simulink library "AFCToolbox2023a"  (R2023a)
settings: Solver=VariableStepAuto  StartTime=0.0  StopTime=10.0  RelTol=1e-3
undefined symbols (not defined in the file or in its folder): AFC5Toolbox_SimuMoudle, AFCToolbox, ax, ay, az, btnSample, C_d, C_dm, C_m, C_t, Control, d, declination_table, dp0, dp1, dp2, dp3, dt, euler_0, g0, I_xyz, inclination_table, J_m, lmd_high, lmd_low, lp_acc_knoise, lp_acc_max, lp_acc_min, lp_acc_seed, lp_GPS_BL_max, lp_GPS_BL_min, lp_GPS_H_max, lp_GPS_H_min, lp_GPS_knoise, lp_GPS_seed, lp_GPS_vel_max, lp_GPS_vel_min, lp_gyro_knoise, lp_gyro_max, lp_gyro_min, lp_gyro_seed, lp_hf_vwind, lp_hs_vwind_interp, lp_kaerorho, lp_kaeroT, lp_kIxyz, lp_kmass, lp_momentx_A0, lp_momentx_Af, lp_momentx_ts, lp_momenty_A0, lp_momenty_Af, lp_momenty_ts, lp_momentz_A0, lp_momentz_Af, lp_momentz_ts, lp_vf_vwind, lp_vs_vwind_interp, lp_vwind_thetax, lp_vwind_thetaz ... (+54)
libraries: $bdroot x104, simulink x75, etargetslib x32, sharedtransform x13, simulink_extras x12, dspstat3 x11, aerolibconvert2 x9, aerolibtransform2 x3, aerolibutil x2, matrix_library x1
(part 7 of 10)

== system AFCToolbox2023a/SimuMoudle/Forces & Moments1/Parameters/Air Parameter1/Air Model/Pressure xishu ==
  note: 9
  note: 1
  note: 2
  note: 3
  note: 4
  note: 5
  note: 6
  note: 7
  note: 8
  Z : Inport
  H : Inport  Port=2
  1 : Switch  Threshold=11.0191  SaturateOnIntegerOverflow=off  InputSameDT=off
  2 : Switch  Threshold=20.0631  SaturateOnIntegerOverflow=off  InputSameDT=off
  3 : Switch  Threshold=32.1619  SaturateOnIntegerOverflow=off  InputSameDT=off
  4 : Switch  Threshold=47.3501  SaturateOnIntegerOverflow=off  InputSameDT=off
  5 : Switch  Threshold=51.4125  SaturateOnIntegerOverflow=off  InputSameDT=off
  6 : Switch  Threshold=71.8020  SaturateOnIntegerOverflow=off  InputSameDT=off
  7 : Switch  Threshold=86  SaturateOnIntegerOverflow=off  InputSameDT=off
  8 : Switch  Threshold=91  SaturateOnIntegerOverflow=off  InputSameDT=off
  Gain : Gain  Gain=1.042e-3
  Gain1 : Gain  Gain=1e-6
  Sum : Sum  Inputs=|++
  constant1 : Constant  Value=2.1671e-4
  constant10 : Constant  Value=8.9155e-4
  constant11 : Constant  Value=2.8338e-3
  constant2 : Constant  Value=0
  constant4 : Constant  Value=1.2274e-5
  constant6 : Constant  Value=2.2730
  constant7 : Constant
  constant8 : Constant  Value=1.1953e-1
  constant9 : Constant  Value=2.5158e-2
  xishu : Outport
  wires:
  Gain1/1 -> 7/1
  Gain/1 -> Sum/2
  H/1 -> Gain/1
  Sum/1 -> Gain1/1
  constant6/1 -> Sum/1
  8/1 -> xishu/1
  7/1 -> 8/3
  constant2/1 -> 8/1
  constant7/1 -> 1/3
  constant8/1 -> 1/1
  constant9/1 -> 2/1
  1/1 -> 2/3
  constant11/1 -> 3/1
  2/1 -> 3/3
  constant10/1 -> 4/1
  3/1 -> 4/3
  constant1/1 -> 5/1
  4/1 -> 5/3
  constant4/1 -> 6/1
  5/1 -> 6/3
  6/1 -> 7/3
  Z/1 -> 2/2, 8/2, 7/2, 6/2, 5/2, 1/2, 3/2, 4/2

== system AFCToolbox2023a/SimuMoudle/Forces & Moments1/Parameters/Air Parameter1/Air Model/T ==
  note: 1
  note: 2
  note: 3
  note: 4
  note: 5
  note: 6
  note: 7
  note: 8
  Z : Inport
  T xishu : Inport  Port=2
  W : Inport  Port=3
  1 : Switch  Threshold=11.0191  SaturateOnIntegerOverflow=off  InputSameDT=off
  2 : Switch  Threshold=20.0631  SaturateOnIntegerOverflow=off  InputSameDT=off
  3 : Switch  Threshold=32.1619  SaturateOnIntegerOverflow=off  InputSameDT=off
  4 : Switch  Threshold=47.3501  SaturateOnIntegerOverflow=off  InputSameDT=off
  5 : Switch  Threshold=51.4125  SaturateOnIntegerOverflow=off  InputSameDT=off
  6 : Switch  Threshold=71.8020  SaturateOnIntegerOverflow=off  InputSameDT=off
  7 : Switch  Threshold=86  SaturateOnIntegerOverflow=off  InputSameDT=off
  Product : Product  RndMeth=Zero
  constant10 : Constant
  constant6 : Constant
  constant8 : Constant
  T : Outport
  wires:
  Product/1 -> T/1
  T xishu/1 -> Product/2
  7/1 -> Product/1
  W/1 -> 3/1, 2/1, 5/1, 6/1, 1/3
  constant8/1 -> 1/1
  1/1 -> 2/3
  2/1 -> 3/3
  constant10/1 -> 4/1
  3/1 -> 4/3
  4/1 -> 5/3
  5/1 -> 6/3
  constant6/1 -> 7/1
  6/1 -> 7/3
  Z/1 -> 2/2, 6/2, 7/2, 5/2, 1/2, 3/2, 4/2

== system AFCToolbox2023a/SimuMoudle/Forces & Moments1/Parameters/Air Parameter1/Air Model/T xishu ==
  note: 8
  note: 7
  note: 6
  note: 5
  note: 4
  note: 3
  note: 2
  note: 1
  Z : Inport
  1 : Switch  Threshold=11.0191  SaturateOnIntegerOverflow=off  InputSameDT=off
  2 : Switch  Threshold=20.0631  SaturateOnIntegerOverflow=off  InputSameDT=off
  3 : Switch  Threshold=32.1619  SaturateOnIntegerOverflow=off  InputSameDT=off
  4 : Switch  Threshold=47.3501  SaturateOnIntegerOverflow=off  InputSameDT=off
  5 : Switch  Threshold=51.4125  SaturateOnIntegerOverflow=off  InputSameDT=off
  6 : Switch  Threshold=71.8020  SaturateOnIntegerOverflow=off  InputSameDT=off
  7 : Switch  Threshold=86  SaturateOnIntegerOverflow=off  InputSameDT=off
  constant1 : Constant  Value=247.021
  constant10 : Constant  Value=270.650
  constant11 : Constant  Value=250.350
  constant4 : Constant  Value=200.590
  constant6 : Constant  Value=186.870
  constant7 : Constant  Value=288.15
  constant8 : Constant  Value=216.650
  constant9 : Constant  Value=221.552
  T xishu : Outport
  wires:
  7/1 -> T xishu/1
  Z/1 -> 4/2, 3/2, 1/2, 5/2, 7/2, 6/2, 2/2
  6/1 -> 7/3
  constant6/1 -> 7/1
  5/1 -> 6/3
  constant4/1 -> 6/1
  4/1 -> 5/3
  constant1/1 -> 5/1
  3/1 -> 4/3
  constant10/1 -> 4/1
  2/1 -> 3/3
  constant11/1 -> 3/1
  1/1 -> 2/3
  constant9/1 -> 2/1
  constant8/1 -> 1/1
  constant7/1 -> 1/3

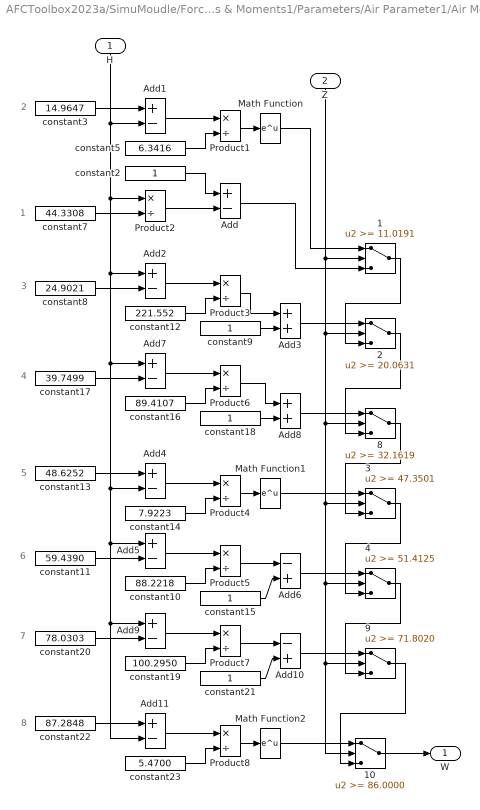
== system AFCToolbox2023a/SimuMoudle/Forces & Moments1/Parameters/Air Parameter1/Air Model/W ==
  note: 8
  note: 7
  note: 4
  note: 6
  note: 5
  note: 3
  note: 2
  note: 1
  H : Inport
  Z : Inport  Port=2
  1 : Switch  Threshold=11.0191  SaturateOnIntegerOverflow=off  InputSameDT=off
  10 : Switch  Threshold=86.0000  SaturateOnIntegerOverflow=off  InputSameDT=off
  2 : Switch  Threshold=20.0631  SaturateOnIntegerOverflow=off  InputSameDT=off
  3 : Switch  Threshold=47.3501  SaturateOnIntegerOverflow=off  InputSameDT=off
  4 : Switch  Threshold=51.4125  SaturateOnIntegerOverflow=off  InputSameDT=off
  8 : Switch  Threshold=32.1619  SaturateOnIntegerOverflow=off  InputSameDT=off
  9 : Switch  Threshold=71.8020  SaturateOnIntegerOverflow=off  InputSameDT=off
  Add{,1..2,4..5,7,9,11} (8 alike) : Sum  Inputs=+-
  Add10 : Sum  Inputs=-+
  Add3 : Sum  Inputs=2
  Add6 : Sum  Inputs=-+
  Add8 : Sum  Inputs=2
  Math Function : Math  SignedPower=on
  Math Function1 : Math  SignedPower=on
  Math Function2 : Math  SignedPower=on
  Product{1..8} (8 alike) : Product  Inputs=*/  RndMeth=Zero
  constant10 : Constant  Value=88.2218
  constant11 : Constant  Value=59.4390
  constant12 : Constant  Value=221.552
  constant13 : Constant  Value=48.6252
  constant14 : Constant  Value=7.9223
  constant{2,9,15,18,21} (5 alike) : Constant
  constant16 : Constant  Value=89.4107
  constant17 : Constant  Value=39.7499
  constant19 : Constant  Value=100.2950
  constant20 : Constant  Value=78.0303
  constant22 : Constant  Value=87.2848
  constant23 : Constant  Value=5.4700
  constant3 : Constant  Value=14.9647
  constant5 : Constant  Value=6.3416
  constant7 : Constant  Value=44.3308
  constant8 : Constant  Value=24.9021
  W : Outport
  wires:
  Z/1 -> 1/2, 2/2, 8/2, 3/2, 4/2, 9/2, 10/2
  10/1 -> W/1
  9/1 -> 10/3
  constant22/1 -> Add11/1
  Math Function2/1 -> 10/1
  Product8/1 -> Math Function2/1
  constant23/1 -> Product8/2
  Add11/1 -> Product8/1
  Add10/1 -> 9/1
  constant21/1 -> Add10/2
  Product7/1 -> Add10/1
  constant20/1 -> Add9/2
  constant19/1 -> Product7/2
  Add9/1 -> Product7/1
  4/1 -> 9/3
  Add7/1 -> Product6/1
  8/1 -> 3/3
  Add8/1 -> 8/1
  constant18/1 -> Add8/2
  Product6/1 -> Add8/1
  constant17/1 -> Add7/2
  constant16/1 -> Product6/2
  2/1 -> 8/3
  Add6/1 -> 4/1
  constant15/1 -> Add6/2
  Product5/1 -> Add6/1
  constant11/1 -> Add5/2
  constant10/1 -> Product5/2
  Add5/1 -> Product5/1
  Math Function1/1 -> 3/1
  Product4/1 -> Math Function1/1
  constant14/1 -> Product4/2
  Add4/1 -> Product4/1
  constant13/1 -> Add4/1
  Add3/1 -> 2/1
  constant9/1 -> Add3/2
  Product3/1 -> Add3/1
  constant8/1 -> Add2/2
  constant12/1 -> Product3/2
  Add2/1 -> Product3/1
  Math Function/1 -> 1/1
  Product1/1 -> Math Function/1
  constant5/1 -> Product1/2
  Add1/1 -> Product1/1
  constant3/1 -> Add1/1
  Product2/1 -> Add/2
  constant2/1 -> Add/1
  constant7/1 -> Product2/2
  Add/1 -> 1/3
  1/1 -> 2/3
  3/1 -> 4/3
  H/1 -> Add7/1, Add11/2, Add9/1, Add5/1, Add4/2, Add2/1, Product2/1, Add1/2

== system AFCToolbox2023a/SimuMoudle/Forces & Moments1/Parameters/Air Parameter1/Air Model/W zhishu ==
  note: 1
  note: 2
  note: 3
  note: 4
  note: 5
  note: 6
  note: 7
  note: 8
  Z : Inport
  1 : Switch  Threshold=11.0191  SaturateOnIntegerOverflow=off  InputSameDT=off
  2 : Switch  Threshold=20.0631  SaturateOnIntegerOverflow=off  InputSameDT=off
  3 : Switch  Threshold=32.1619  SaturateOnIntegerOverflow=off  InputSameDT=off
  4 : Switch  Threshold=47.3501  SaturateOnIntegerOverflow=off  InputSameDT=off
  5 : Switch  Threshold=51.4125  SaturateOnIntegerOverflow=off  InputSameDT=off
  6 : Switch  Threshold=71.8020  SaturateOnIntegerOverflow=off  InputSameDT=off
  7 : Switch  Threshold=86  SaturateOnIntegerOverflow=off  InputSameDT=off
  constant1 : Constant  Value=11.2011
  constant10 : Constant
  constant11 : Constant  Value=-13.2011
  constant4 : Constant  Value=16.0816
  constant6 : Constant
  constant7 : Constant  Value=4.2559
  constant8 : Constant
  constant9 : Constant  Value=-35.1629
  zhishu : Outport
  wires:
  constant7/1 -> 1/3
  constant8/1 -> 1/1
  constant9/1 -> 2/1
  1/1 -> 2/3
  constant11/1 -> 3/1
  2/1 -> 3/3
  constant10/1 -> 4/1
  3/1 -> 4/3
  constant1/1 -> 5/1
  4/1 -> 5/3
  constant4/1 -> 6/1
  5/1 -> 6/3
  constant6/1 -> 7/1
  6/1 -> 7/3
  Z/1 -> 2/2, 6/2, 7/2, 5/2, 1/2, 3/2, 4/2
  7/1 -> zhishu/1

== system AFCToolbox2023a/SimuMoudle/Forces & Moments1/Parameters/Air Parameter1/Air Model/W zhishu1 ==
  note: 8
  note: 7
  note: 6
  note: 5
  note: 4
  note: 3
  note: 2
  note: 1
  Z : Inport
  1 : Switch  Threshold=11.0191  SaturateOnIntegerOverflow=off  InputSameDT=off
  2 : Switch  Threshold=20.0631  SaturateOnIntegerOverflow=off  InputSameDT=off
  3 : Switch  Threshold=32.1619  SaturateOnIntegerOverflow=off  InputSameDT=off
  4 : Switch  Threshold=47.3501  SaturateOnIntegerOverflow=off  InputSameDT=off
  5 : Switch  Threshold=51.4125  SaturateOnIntegerOverflow=off  InputSameDT=off
  6 : Switch  Threshold=71.8020  SaturateOnIntegerOverflow=off  InputSameDT=off
  7 : Switch  Threshold=86  SaturateOnIntegerOverflow=off  InputSameDT=off
  constant1 : Constant  Value=12.2011
  constant10 : Constant
  constant11 : Constant  Value=-12.2011
  constant4 : Constant  Value=17.0816
  constant6 : Constant
  constant7 : Constant  Value=5.2559
  constant8 : Constant
  constant9 : Constant  Value=-34.1629
  zhishu : Outport
  wires:
  7/1 -> zhishu/1
  Z/1 -> 4/2, 3/2, 1/2, 5/2, 7/2, 6/2, 2/2
  6/1 -> 7/3
  constant6/1 -> 7/1
  5/1 -> 6/3
  constant4/1 -> 6/1
  4/1 -> 5/3
  constant1/1 -> 5/1
  3/1 -> 4/3
  constant10/1 -> 4/1
  2/1 -> 3/3
  constant11/1 -> 3/1
  1/1 -> 2/3
  constant9/1 -> 2/1
  constant8/1 -> 1/1
  constant7/1 -> 1/3

== system AFCToolbox2023a/SimuMoudle/Forces & Moments1/Parameters/Air Parameter1/Air Model/rho xishu ==
  note: 8
  note: 7
  note: 6
  note: 5
  note: 4
  note: 3
  note: 2
  note: 1
  note: 9
  Z : Inport
  1 : Switch  Threshold=11.0191  SaturateOnIntegerOverflow=off  InputSameDT=off
  2 : Switch  Threshold=20.0631  SaturateOnIntegerOverflow=off  InputSameDT=off
  3 : Switch  Threshold=32.1619  SaturateOnIntegerOverflow=off  InputSameDT=off
  4 : Switch  Threshold=47.3501  SaturateOnIntegerOverflow=off  InputSameDT=off
  5 : Switch  Threshold=51.4125  SaturateOnIntegerOverflow=off  InputSameDT=off
  6 : Switch  Threshold=71.8020  SaturateOnIntegerOverflow=off  InputSameDT=off
  7 : Switch  Threshold=86  SaturateOnIntegerOverflow=off  InputSameDT=off
  8 : Switch  Threshold=91  SaturateOnIntegerOverflow=off  InputSameDT=off
  constant1 : Constant  Value=2.5280e-4
  constant10 : Constant  Value=9.4920e-4
  constant11 : Constant  Value=3.2618e-3
  constant2 : Constant  Value=0
  constant4 : Constant  Value=1.7632e-5
  constant6 : Constant  Value=3.6411e-6
  constant7 : Constant
  constant8 : Constant  Value=1.5898e-1
  constant9 : Constant  Value=3.2722e-2
  xishu : Outport
  wires:
  Z/1 -> 4/2, 3/2, 1/2, 5/2, 6/2, 7/2, 8/2, 2/2
  6/1 -> 7/3
  constant6/1 -> 7/1
  5/1 -> 6/3
  constant4/1 -> 6/1
  4/1 -> 5/3
  constant1/1 -> 5/1
  3/1 -> 4/3
  constant10/1 -> 4/1
  2/1 -> 3/3
  constant11/1 -> 3/1
  1/1 -> 2/3
  constant9/1 -> 2/1
  constant8/1 -> 1/1
  constant7/1 -> 1/3
  constant2/1 -> 8/1
  7/1 -> 8/3
  8/1 -> xishu/1

== system AFCToolbox2023a/SimuMoudle/Position-Control/Leader/Subsystem/Follower1/Subsystem ==
  v111_k_1 : Inport
  v000_k_1 : Inport  Port=2
  Abs : Abs  SaturateOnIntegerOverflow=off
  Abs1 : Abs  SaturateOnIntegerOverflow=off
  Abs2 : Abs  SaturateOnIntegerOverflow=off
  Add : Sum  Inputs=+-
  Add1 : Sum  Inputs=+-
  Add2 : Sum  Inputs=+-
  Demux : Demux  Outputs=3
  Demux1 : Demux  Outputs=3
  Max : MinMax  Function=max  Inputs=3
  Relational Operator : RelationalOperator  Operator=>  OutDataTypeStr=boolean  RndMeth=Simplest  InputSameDT=off
  get lmd : Subsystem
  order : Outport
  wires:
  Relational Operator/1 -> order/1
  get lmd/1(lmd) -> Relational Operator/2
  Max/1 -> Relational Operator/1
  Abs2/1 -> Max/3
  Abs1/1 -> Max/2
  Abs/1 -> Max/1
  Add2/1 -> Abs2/1
  Add1/1 -> Abs1/1
  Add/1 -> Abs/1
  Demux/3 -> Add2/1
  Demux1/3 -> Add2/2
  Demux1/2 -> Add1/2
  Demux/2 -> Add1/1
  Demux1/1 -> Add/2
  Demux/1 -> Add/1
  v000_k_1/1 -> Demux1/1
  v111_k_1/1 -> Demux/1

== system AFCToolbox2023a/SimuMoudle/Position-Control/Leader/Subsystem/Follower1/Subsystem1 ==
  Clock : Clock
  Constant : Constant
  Constant1 : Constant  Value=0
  Switch1 : Switch  Criteria=u2 > Threshold  Threshold=40  SaturateOnIntegerOverflow=off  InputSameDT=off
  Out1 : Outport
  wires:
  Switch1/1 -> Out1/1
  Constant1/1 -> Switch1/3
  Constant/1 -> Switch1/1
  Clock/1 -> Switch1/2

== system AFCToolbox2023a/SimuMoudle/Position-Control/Leader/Subsystem/Follower1/质心运动方程 ==
  v1 : Inport
  theta1 : Inport  Port=2
  phi1 : Inport  Port=3
  Enable : EnablePort
  Cos : Trigonometry  Operator=cos
  Cos1 : Trigonometry  Operator=cos
  Mux : Mux  Inputs=3
  Product : Product  Inputs=3
  Product1 : Product  Inputs=3
  Product2 : Product
  Sin : Trigonometry
  Sin1 : Trigonometry
  v111 : Outport
  wires:
  theta1/1 -> Cos/1, Sin/1
  phi1/1 -> Cos1/1, Sin1/1
  Cos/1 -> Product/1
  v1/1 -> Product2/2, Product1/3, Product/3
  Product/1 -> Mux/1
  Product1/1 -> Mux/2
  Sin/1 -> Product1/1
  Cos1/1 -> Product/2, Product1/2
  Product2/1 -> Mux/3
  Mux/1 -> v111/1
  Sin1/1 -> Product2/1

== system AFCToolbox2023a/SimuMoudle/Position-Control/Leader/Subsystem/Follower2/Subsystem ==
  v222_k_1 : Inport
  v000_k_1 : Inport  Port=2
  Abs : Abs  SaturateOnIntegerOverflow=off
  Abs1 : Abs  SaturateOnIntegerOverflow=off
  Abs2 : Abs  SaturateOnIntegerOverflow=off
  Add : Sum  Inputs=+-
  Add1 : Sum  Inputs=+-
  Add2 : Sum  Inputs=+-
  Demux : Demux  Outputs=3
  Demux1 : Demux  Outputs=3
  Max : MinMax  Function=max  Inputs=3
  Relational Operator : RelationalOperator  Operator=>  OutDataTypeStr=boolean  RndMeth=Simplest  InputSameDT=off
  get lmd : Subsystem
  order : Outport
  wires:
  v222_k_1/1 -> Demux/1
  v000_k_1/1 -> Demux1/1
  Demux/1 -> Add/1
  Demux1/1 -> Add/2
  Demux/2 -> Add1/1
  Demux1/2 -> Add1/2
  Demux1/3 -> Add2/2
  Demux/3 -> Add2/1
  Add/1 -> Abs/1
  Add1/1 -> Abs1/1
  Add2/1 -> Abs2/1
  Abs/1 -> Max/1
  Abs1/1 -> Max/2
  Abs2/1 -> Max/3
  Max/1 -> Relational Operator/1
  get lmd/1(lmd) -> Relational Operator/2
  Relational Operator/1 -> order/1

== system AFCToolbox2023a/SimuMoudle/Position-Control/Leader/Subsystem/Follower2/Subsystem1 ==
  Clock : Clock
  Constant : Constant
  Constant1 : Constant  Value=0
  Switch1 : Switch  Criteria=u2 > Threshold  Threshold=40  SaturateOnIntegerOverflow=off  InputSameDT=off
  Out1 : Outport
  wires:
  Switch1/1 -> Out1/1
  Constant1/1 -> Switch1/3
  Constant/1 -> Switch1/1
  Clock/1 -> Switch1/2

== system AFCToolbox2023a/SimuMoudle/Position-Control/Leader/Subsystem/Follower2/质心运动方程 ==
  v2 : Inport
  theta2 : Inport  Port=2
  phi2 : Inport  Port=3
  Enable : EnablePort
  Cos : Trigonometry  Operator=cos
  Cos1 : Trigonometry  Operator=cos
  Mux : Mux  Inputs=3
  Product : Product  Inputs=3
  Product1 : Product  Inputs=3
  Product2 : Product
  Sin : Trigonometry
  Sin1 : Trigonometry
  v222 : Outport
  wires:
  Sin1/1 -> Product2/1
  Mux/1 -> v222/1
  Product2/1 -> Mux/3
  Cos1/1 -> Product1/2, Product/2
  Sin/1 -> Product1/1
  Product1/1 -> Mux/2
  Product/1 -> Mux/1
  v2/1 -> Product/3, Product1/3, Product2/2
  Cos/1 -> Product/1
  phi2/1 -> Sin1/1, Cos1/1
  theta2/1 -> Sin/1, Cos/1

== system AFCToolbox2023a/SimuMoudle/Position-Control/Leader/Subsystem/Follower3/Subsystem ==
  v333_k_1 : Inport
  v000_k_1 : Inport  Port=2
  Abs : Abs  SaturateOnIntegerOverflow=off
  Abs1 : Abs  SaturateOnIntegerOverflow=off
  Abs2 : Abs  SaturateOnIntegerOverflow=off
  Add : Sum  Inputs=+-
  Add1 : Sum  Inputs=+-
  Add2 : Sum  Inputs=+-
  Demux : Demux  Outputs=3
  Demux1 : Demux  Outputs=3
  Max : MinMax  Function=max  Inputs=3
  Relational Operator : RelationalOperator  Operator=>  OutDataTypeStr=boolean  RndMeth=Simplest  InputSameDT=off
  get lmd : Subsystem
  order : Outport
  wires:
  Relational Operator/1 -> order/1
  get lmd/1(lmd) -> Relational Operator/2
  Max/1 -> Relational Operator/1
  Abs2/1 -> Max/3
  Abs1/1 -> Max/2
  Abs/1 -> Max/1
  Add2/1 -> Abs2/1
  Add1/1 -> Abs1/1
  Add/1 -> Abs/1
  Demux/3 -> Add2/1
  Demux1/3 -> Add2/2
  Demux1/2 -> Add1/2
  Demux/2 -> Add1/1
  Demux1/1 -> Add/2
  Demux/1 -> Add/1
  v000_k_1/1 -> Demux1/1
  v333_k_1/1 -> Demux/1

== system AFCToolbox2023a/SimuMoudle/Position-Control/Leader/Subsystem/Follower3/Subsystem1 ==
  Clock : Clock
  Constant : Constant
  Constant1 : Constant  Value=0
  Switch1 : Switch  Criteria=u2 > Threshold  Threshold=40  SaturateOnIntegerOverflow=off  InputSameDT=off
  Out1 : Outport
  wires:
  Switch1/1 -> Out1/1
  Constant1/1 -> Switch1/3
  Constant/1 -> Switch1/1
  Clock/1 -> Switch1/2

== system AFCToolbox2023a/SimuMoudle/Position-Control/Leader/Subsystem/Follower3/质心运动方程 ==
  v3 : Inport
  theta3 : Inport  Port=2
  phi3 : Inport  Port=3
  Enable : EnablePort
  Cos : Trigonometry  Operator=cos
  Cos1 : Trigonometry  Operator=cos
  Mux : Mux  Inputs=3
  Product : Product  Inputs=3
  Product1 : Product  Inputs=3
  Product2 : Product
  Sin : Trigonometry
  Sin1 : Trigonometry
  v333 : Outport
  wires:
  theta3/1 -> Cos/1, Sin/1
  phi3/1 -> Cos1/1, Sin1/1
  Cos/1 -> Product/1
  v3/1 -> Product2/2, Product1/3, Product/3
  Product/1 -> Mux/1
  Product1/1 -> Mux/2
  Sin/1 -> Product1/1
  Cos1/1 -> Product/2, Product1/2
  Product2/1 -> Mux/3
  Mux/1 -> v333/1
  Sin1/1 -> Product2/1

== system AFCToolbox2023a/SimuMoudle/UAV/Forces & Moments/Moments/Disturb/Dist Mx ==
  N : Inport
  Step2 : Step  Time=ts_0  Before=A0  After=Af
  Sum : Sum  Inputs=|++
  D : Outport
  wires:
  Sum/1 -> D/1
  N/1 -> Sum/1
  Step2/1 -> Sum/2

== system AFCToolbox2023a/SimuMoudle/UAV/Forces & Moments/Moments/Disturb/Dist My ==
  N : Inport
  Step2 : Step  Time=ts_0  Before=A0  After=Af
  Sum : Sum  Inputs=|++
  D : Outport
  wires:
  Step2/1 -> Sum/2
  N/1 -> Sum/1
  Sum/1 -> D/1

== system AFCToolbox2023a/SimuMoudle/UAV/Forces & Moments/Moments/Disturb/Dist Mz ==
  N : Inport
  Step2 : Step  Time=ts_0  Before=A0  After=Af
  Sum : Sum  Inputs=|++
  D : Outport
  wires:
  Sum/1 -> D/1
  N/1 -> Sum/1
  Step2/1 -> Sum/2

== system AFCToolbox2023a/SimuMoudle/UAV/Forces & Moments/Parameters/Air Parameter1/Air Model ==
  note: rho
  v : Inport
  h (km) : Inport  Port=2
  1/2 : Constant  Value=0.5
  Gain lp_kaeroT : Gain  Gain=lp_kaeroT
  Gain lp_kaerorho : Gain  Gain=lp_kaerorho
  H : Subsystem
      mask Display: disp('h --> H')
  Math Function : Math  Operator=sqrt  SignedPower=on
  Math Function1 : Math  Operator=pow  SignedPower=on
  Math Function2 : Math  Operator=pow  SignedPower=on
  PSL : Constant  Value=101325
  Pressure xishu : Subsystem
  Product : Product  Inputs=/*  SaturateOnIntegerOverflow=on  OutDataTypeStr=Inherit: Same as first input
  Product1 : Product  RndMeth=Zero
  Product2 : Product  Inputs=3  RndMeth=Zero
  Product3 : Product  Inputs=4  RndMeth=Zero
  Product4 : Product  Inputs=3  RndMeth=Zero
  T : Subsystem
  T xishu : Subsystem
  W : Subsystem
  W zhishu : Subsystem
  W zhishu1 : Subsystem
  constant2 : Constant  Value=20.0468
  rho xishu : Subsystem
  rhoSL : Constant  Value=1.225
  dongYaTou : Outport
  Mach : Outport  Port=2
  Pressure : Outport  Port=3
  wires:
  Product4/1 -> Pressure/1
  PSL/1 -> Product4/3
  Math Function2/1 -> Product4/1
  Pressure xishu/1(xishu) -> Product4/2
  W zhishu1/1(zhishu) -> Math Function2/2
  Gain lp_kaerorho/1 -> Product3/4
  Gain lp_kaeroT/1 -> Math Function/1
  v/1 -> Product3/1, Product/2, Product3/2
  Product/1 -> Mach/1
  Product1/1 -> Product/1
  1/2/1 -> Product3/3
  T/1(T) -> Gain lp_kaeroT/1
  h (km)/1 -> H/1(h), T/1(Z), Pressure xishu/1(Z), W zhishu1/1(Z), rho xishu/1(Z), W zhishu/1(Z), W/2(Z), T xishu/1(Z)
  H/1(H) -> Pressure xishu/2(H), W/1(H)
  W zhishu/1(zhishu) -> Math Function1/2
  Product3/1 -> dongYaTou/1
  Product2/1 -> Gain lp_kaerorho/1
  rhoSL/1 -> Product2/3
  rho xishu/1(xishu) -> Product2/2
  Math Function1/1 -> Product2/1
  W/1(W) -> Math Function2/1, Math Function1/1, T/3(W)
  T xishu/1(T xishu) -> T/2(T xishu)
  constant2/1 -> Product1/2
  Math Function/1 -> Product1/1

== system AFCToolbox2023a/SimuMoudle/UAV/Forces & Moments/Parameters/Wind Velocity/Vector ==
  abs : Inport
  thetaz : Inport  Port=2
  thetax : Inport  Port=3
  Mux : Mux  Inputs=3
  Selector : Selector  InputPortWidth=3  IndexOptions=Index vector (dialog)  Indices=[3 2 1]  OutputSizes=1
  sin thetax cos thetax : Trigonometry  Operator=sincos
  sin thetaz cos thetaz : Trigonometry  Operator=sincos
  vwind cos z : Product  RndMeth=Zero
  vwind sin z : Product  RndMeth=Zero
  vwind xy cos x : Product  RndMeth=Zero
  vwind xy sin x : Product  RndMeth=Zero
  xyz : Outport
  wires:
  abs/1 -> vwind cos z/1, vwind sin z/1
  sin thetaz cos thetaz/1 -> vwind sin z/2
  sin thetaz cos thetaz/2 -> vwind cos z/2
  vwind sin z/1 -> Mux/1
  sin thetax cos thetax/1 -> vwind xy sin x/2
  sin thetax cos thetax/2 -> vwind xy cos x/2
  vwind cos z/1 -> vwind xy cos x/1, vwind xy sin x/1
  vwind xy cos x/1 -> Mux/3
  vwind xy sin x/1 -> Mux/2
  Mux/1 -> Selector/1
  thetaz/1 -> sin thetaz cos thetaz/1
  Selector/1 -> xyz/1
  thetax/1 -> sin thetax cos thetax/1

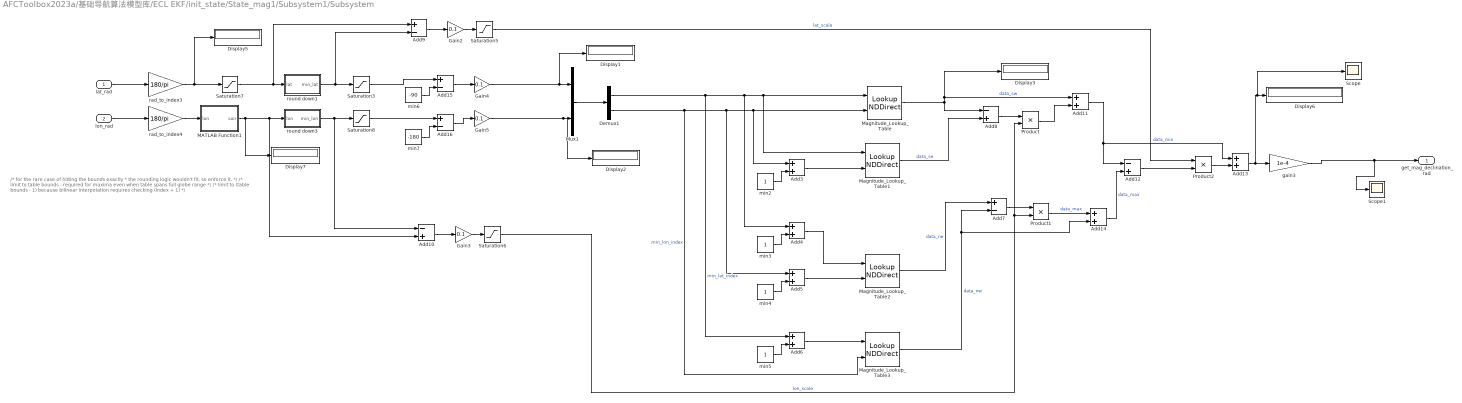
== system AFCToolbox2023a/基础导航算法模型库/ECL EKF/init_state/State_mag1/Subsystem1/Subsystem ==
  note: /* for the rare case of hitting the bounds exactly
      | 	 * the rounding logic wouldn't fit, so enforce it. */
      |
      | 	/* limit to table bounds - required for maxima even when table spans full globe range */
      | 	/* limit to (table bounds - 1) because bilinear interpolation requires checking (index + 1) */
  lat_rad : Inport
  lon_rad : Inport  Port=2
  Add10 : Sum  Inputs=-+
  Add{3..6,11,13..14} (7 alike) : Sum
  Add12 : Sum  Inputs=-+
  Add{7,9,15..16} (4 alike) : Sum  Inputs=+-
  Add8 : Sum  Inputs=-+
  Demux1 : Demux  Outputs=2
  Display{1..3,5..7} (6 alike) : Display
      Display6 settings: Decimation=4
  Gain{2..5} (4 alike) : Gain  Gain=0.1
  MATLAB Function1 : MATLAB Function  TreatAsAtomicUnit=on
  Magnitude_Lookup_Table{,1..3} (4 alike) : LookupNDDirect  Table=declination_table  DiagnosticForOutOfRangeInput=Error
  Mux1 : Mux  Inputs=2
  Product : Product
  Product1 : Product
  Product2 : Product
  Saturation3 : Saturate  UpperLimit=80  LowerLimit=-90
  Saturation5 : Saturate  UpperLimit=1  LowerLimit=0
  Saturation6 : Saturate  UpperLimit=1  LowerLimit=0
  Saturation7 : Saturate  UpperLimit=90  LowerLimit=-90
  Saturation8 : Saturate  UpperLimit=170  LowerLimit=-180
  Scope : Scope
  Scope1 : Scope
  gain3 : Gain  Gain=1e-4
  min{2..5} (4 alike) : Constant
  min6 : Constant  Value=-90
  min7 : Constant  Value=-180
  rad_to_index3 : Gain  Gain=180/pi  OutDataTypeStr=int32
  rad_to_index4 : Gain  Gain=180/pi  OutDataTypeStr=int32
  round down1 : Subsystem
  round down3 : Subsystem
  get_mag_declination_rad : Outport
  wires:
  Magnitude_Lookup_Table1/1 -> Add8/2  "data_se"
  Demux1/1 -> Magnitude_Lookup_Table/1, Magnitude_Lookup_Table1/1, Add4/1, Add6/1  "min_lat_index"
  Product1/1 -> Add14/1  "data_max"
  Magnitude_Lookup_Table/1 -> Add8/1, Display3/1, Add11/1  "data_sw"
  Demux1/2 -> Magnitude_Lookup_Table3/2, Magnitude_Lookup_Table/2, Add3/1, Add5/1  "min_lon_index"
  Add8/1 -> Product/1
  Add14/1 -> Add12/2  "data_max"
  Saturation5/1 -> Product2/1  "lat_scale"
  min3/1 -> Add4/2
  Gain3/1 -> Saturation6/1
  Add11/1 -> Add13/1, Add12/1  "data_min"
  Add5/1 -> Magnitude_Lookup_Table2/2
  Add13/1 -> Scope/1, Display6/1, gain3/1
  Product/1 -> Add11/2
  Magnitude_Lookup_Table2/1 -> Add7/1  "data_ne"
  Magnitude_Lookup_Table3/1 -> Add14/2, Add7/2  "data_nw"
  Saturation6/1 -> Product/2, Product1/2  "lon_scale"
  Product2/1 -> Add13/2
  Add3/1 -> Magnitude_Lookup_Table1/2
  Add4/1 -> Magnitude_Lookup_Table2/1
  Add7/1 -> Product1/1
  min5/1 -> Add6/2
  Add12/1 -> Product2/2
  Gain2/1 -> Saturation5/1
  Add10/1 -> Gain3/1
  min2/1 -> Add3/2
  Add9/1 -> Gain2/1
  min4/1 -> Add5/2
  Add6/1 -> Magnitude_Lookup_Table3/1
  Gain5/1 -> Display2/1, Mux1/2
  Mux1/1 -> Demux1/1
  Saturation7/1 -> Add9/1, round down1/1(lat)
  rad_to_index4/1 -> MATLAB Function1/1(lon)
  rad_to_index3/1 -> Display5/1, Saturation7/1
  MATLAB Function1/1(Lon) -> Display7/1, Add10/2, round down3/1(lon)
  round down1/1(min_lat) -> Add9/2, Saturation3/1
  Add15/1 -> Gain4/1
  Gain4/1 -> Display1/1, Mux1/1
  min6/1 -> Add15/2
  Saturation8/1 -> Add16/1
  round down3/1(min_lon) -> Add10/1, Saturation8/1
  Saturation3/1 -> Add15/1
  Add16/1 -> Gain5/1
  min7/1 -> Add16/2
  lon_rad/1 -> rad_to_index4/1
  lat_rad/1 -> rad_to_index3/1
  gain3/1 -> Scope1/1, get_mag_declination_rad/1

== system AFCToolbox2023a/基础导航算法模型库/ECL EKF/init_state/State_mag1/Subsystem1/Subsystem2 ==
  note: /* for the rare case of hitting the bounds exactly
      | 	 * the rounding logic wouldn't fit, so enforce it. */
      |
      | 	/* limit to table bounds - required for maxima even when table spans full globe range */
      | 	/* limit to (table bounds - 1) because bilinear interpolation requires checking (index + 1) */
  lat_rad : Inport
  lon_rad : Inport  Port=2
  Add10 : Sum  Inputs=-+
  Add{3..6,11,13..14} (7 alike) : Sum
  Add12 : Sum  Inputs=-+
  Add{7,9,15..16} (4 alike) : Sum  Inputs=+-
  Add8 : Sum  Inputs=-+
  Demux1 : Demux  Outputs=2
  Display : Display
  Display1 : Display
  Gain{2..5} (4 alike) : Gain  Gain=0.1
  MATLAB Function1 : MATLAB Function  TreatAsAtomicUnit=on
  Magnitude_Lookup_Table{1..4} (4 alike) : LookupNDDirect  Table=strength_table  DiagnosticForOutOfRangeInput=Error
  Mux1 : Mux  Inputs=2
  Product : Product
  Product1 : Product
  Product2 : Product
  Saturation3 : Saturate  UpperLimit=80  LowerLimit=-90
  Saturation5 : Saturate  UpperLimit=1  LowerLimit=-1
  Saturation6 : Saturate  UpperLimit=1  LowerLimit=-1
  Saturation7 : Saturate  UpperLimit=90  LowerLimit=-90
  Saturation8 : Saturate  UpperLimit=170  LowerLimit=-180
  gain3 : Gain  Gain=0.0001
  min{2..5} (4 alike) : Constant
  min6 : Constant  Value=-90
  min7 : Constant  Value=-180
  rad_to_index3 : Gain  Gain=180/pi  OutDataTypeStr=int32
  rad_to_index4 : Gain  Gain=180/pi  OutDataTypeStr=int32
  round down1 : Subsystem
  round down3 : Subsystem
  get_mag_strength_gauss : Outport
  wires:
  lat_rad/1 -> rad_to_index3/1
  lon_rad/1 -> rad_to_index4/1
  min7/1 -> Add16/2
  Add16/1 -> Gain5/1
  Saturation3/1 -> Add15/1
  round down3/1(min_lon) -> Saturation8/1, Add10/1
  Saturation8/1 -> Add16/1
  min6/1 -> Add15/2
  Gain4/1 -> Mux1/1
  Add15/1 -> Gain4/1
  round down1/1(min_lat) -> Saturation3/1, Add9/2
  MATLAB Function1/1(Lon) -> round down3/1(lon), Add10/2
  rad_to_index3/1 -> Saturation7/1
  rad_to_index4/1 -> MATLAB Function1/1(lon)
  Saturation7/1 -> round down1/1(lat), Add9/1
  Mux1/1 -> Demux1/1
  Gain5/1 -> Mux1/2, Display/1
  Add6/1 -> Magnitude_Lookup_Table3/1
  min4/1 -> Add5/2
  gain3/1 -> Display1/1, get_mag_strength_gauss/1
  Add9/1 -> Gain2/1
  min2/1 -> Add3/2
  Add10/1 -> Gain3/1
  Gain2/1 -> Saturation5/1
  Add12/1 -> Product2/2
  min5/1 -> Add6/2
  Add7/1 -> Product1/1
  Add4/1 -> Magnitude_Lookup_Table2/1
  Add3/1 -> Magnitude_Lookup_Table1/2
  Product2/1 -> Add13/2
  Saturation6/1 -> Product/2, Product1/2  "lon_scale"
  Magnitude_Lookup_Table3/1 -> Add7/2, Add14/2  "data_nw"
  Magnitude_Lookup_Table2/1 -> Add7/1  "data_ne"
  Product/1 -> Add11/2
  Add13/1 -> gain3/1
  Add5/1 -> Magnitude_Lookup_Table2/2
  Add11/1 -> Add12/1, Add13/1  "data_min"
  Gain3/1 -> Saturation6/1
  min3/1 -> Add4/2
  Saturation5/1 -> Product2/1  "lat_scale"
  Add14/1 -> Add12/2  "data_max"
  Add8/1 -> Product/1
  Demux1/2 -> Magnitude_Lookup_Table3/2, Add5/1, Magnitude_Lookup_Table4/2, Add3/1  "min_lon_index"
  Magnitude_Lookup_Table4/1 -> Add11/1, Add8/1  "data_sw"
  Product1/1 -> Add14/1  "data_max"
  Demux1/1 -> Add6/1, Add4/1, Magnitude_Lookup_Table1/1, Magnitude_Lookup_Table4/1  "min_lat_index"
  Magnitude_Lookup_Table1/1 -> Add8/2  "data_se"

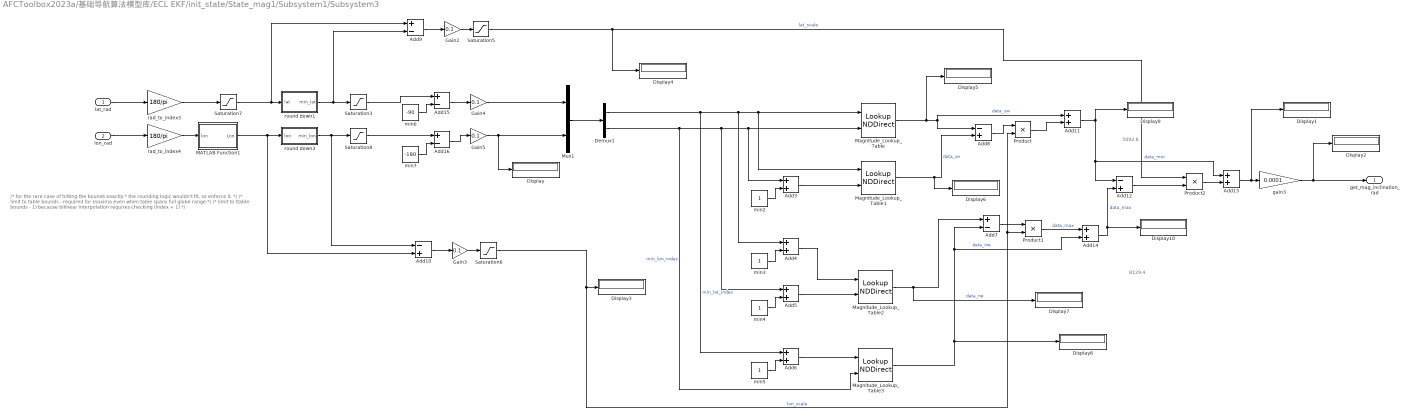
== system AFCToolbox2023a/基础导航算法模型库/ECL EKF/init_state/State_mag1/Subsystem1/Subsystem3 ==
  note: 8129.4
  note: 5092.8
  note: /* for the rare case of hitting the bounds exactly
      | 	 * the rounding logic wouldn't fit, so enforce it. */
      |
      | 	/* limit to table bounds - required for maxima even when table spans full globe range */
      | 	/* limit to (table bounds - 1) because bilinear interpolation requires checking (index + 1) */
  lat_rad : Inport
  lon_rad : Inport  Port=2
  Add10 : Sum  Inputs=-+
  Add{3..6,11,13..14} (7 alike) : Sum
  Add12 : Sum  Inputs=-+
  Add{7,9,15..16} (4 alike) : Sum  Inputs=+-
  Add8 : Sum  Inputs=-+
  Demux1 : Demux  Outputs=2
  Display{,1..10} (11 alike) : Display
  Gain{2..5} (4 alike) : Gain  Gain=0.1
  MATLAB Function1 : MATLAB Function  TreatAsAtomicUnit=on
  Magnitude_Lookup_Table{,1..3} (4 alike) : LookupNDDirect  Table=inclination_table  DiagnosticForOutOfRangeInput=Error
  Mux1 : Mux  Inputs=2
  Product : Product
  Product1 : Product
  Product2 : Product
  Saturation3 : Saturate  UpperLimit=80  LowerLimit=-90
  Saturation5 : Saturate  UpperLimit=1  LowerLimit=-1
  Saturation6 : Saturate  UpperLimit=1  LowerLimit=-1
  Saturation7 : Saturate  UpperLimit=90  LowerLimit=-90
  Saturation8 : Saturate  UpperLimit=170  LowerLimit=-180
  gain3 : Gain  Gain=0.0001
  min{2..5} (4 alike) : Constant
  min6 : Constant  Value=-90
  min7 : Constant  Value=-180
  rad_to_index3 : Gain  Gain=180/pi  OutDataTypeStr=int32
  rad_to_index4 : Gain  Gain=180/pi  OutDataTypeStr=int32
  round down1 : Subsystem
  round down3 : Subsystem
  get_mag_inclination_rad : Outport
  wires:
  lat_rad/1 -> rad_to_index3/1
  lon_rad/1 -> rad_to_index4/1
  min7/1 -> Add16/2
  Add16/1 -> Gain5/1
  Saturation3/1 -> Add15/1
  round down3/1(min_lon) -> Saturation8/1, Add10/1
  Saturation8/1 -> Add16/1
  min6/1 -> Add15/2
  Gain4/1 -> Mux1/1
  Add15/1 -> Gain4/1
  round down1/1(min_lat) -> Saturation3/1, Add9/2
  MATLAB Function1/1(Lon) -> round down3/1(lon), Add10/2
  rad_to_index3/1 -> Saturation7/1
  rad_to_index4/1 -> MATLAB Function1/1(lon)
  Saturation7/1 -> round down1/1(lat), Add9/1
  Mux1/1 -> Demux1/1
  Gain5/1 -> Mux1/2, Display/1
  Add6/1 -> Magnitude_Lookup_Table3/1
  min4/1 -> Add5/2
  gain3/1 -> Display2/1, get_mag_inclination_rad/1
  Add9/1 -> Gain2/1
  min2/1 -> Add3/2
  Add10/1 -> Gain3/1
  Gain2/1 -> Saturation5/1
  Add12/1 -> Product2/2
  min5/1 -> Add6/2
  Add7/1 -> Product1/1
  Add4/1 -> Magnitude_Lookup_Table2/1
  Add3/1 -> Magnitude_Lookup_Table1/2
  Product2/1 -> Add13/2
  Saturation6/1 -> Display3/1, Product/2, Product1/2  "lon_scale"
  Magnitude_Lookup_Table3/1 -> Display8/1, Add7/2, Add14/2  "data_nw"
  Magnitude_Lookup_Table2/1 -> Display7/1, Add7/1  "data_ne"
  Product/1 -> Add11/2
  Add13/1 -> Display1/1, gain3/1
  Add5/1 -> Magnitude_Lookup_Table2/2
  Add11/1 -> Display9/1, Add12/1, Add13/1  "data_min"
  Gain3/1 -> Saturation6/1
  min3/1 -> Add4/2
  Saturation5/1 -> Display4/1, Product2/1  "lat_scale"
  Add14/1 -> Add12/2, Display10/1  "data_max"
  Add8/1 -> Product/1
  Demux1/2 -> Magnitude_Lookup_Table3/2, Add5/1, Add3/1, Magnitude_Lookup_Table/2  "min_lon_index"
  Magnitude_Lookup_Table/1 -> Display5/1, Add11/1, Add8/1  "data_sw"
  Product1/1 -> Add14/1  "data_max"
  Demux1/1 -> Add6/1, Add4/1, Magnitude_Lookup_Table1/1, Magnitude_Lookup_Table/1  "min_lat_index"
  Magnitude_Lookup_Table1/1 -> Display6/1, Add8/2  "data_se"

== system AFCToolbox2023a/SimuMoudle/Position-Control/Leader/Subsystem/Follower1/Subsystem/get lmd ==
  Add : Sum  Inputs=+-
  Add1 : Sum  Inputs=+-
  Gain : Gain  Gain=0.707
  Gain1 : Gain  Gain=0.707
  Min : MinMax  Inputs=2
  lmd high : Constant  Value=lmd_high
  lmd low : Constant  Value=lmd_low
  v0_max : Constant  Value=v0_max
  v0_min : Constant  Value=v0_min
  lmd : Outport
  wires:
  Min/1 -> lmd/1
  Gain1/1 -> Min/2
  Gain/1 -> Min/1
  Add1/1 -> Gain1/1
  lmd high/1 -> Add1/1
  v0_max/1 -> Add1/2
  Add/1 -> Gain/1
  lmd low/1 -> Add/2
  v0_min/1 -> Add/1

== system AFCToolbox2023a/SimuMoudle/Position-Control/Leader/Subsystem/Follower2/Subsystem/get lmd ==
  Add : Sum  Inputs=+-
  Add1 : Sum  Inputs=+-
  Gain : Gain  Gain=0.707
  Gain1 : Gain  Gain=0.707
  Min : MinMax  Inputs=2
  lmd high : Constant  Value=6.45
  lmd low : Constant  Value=0.45
  v0_max : Constant  Value=3.5
  v0_min : Constant  Value=3
  lmd : Outport
  wires:
  v0_min/1 -> Add/1
  lmd low/1 -> Add/2
  Add/1 -> Gain/1
  v0_max/1 -> Add1/2
  lmd high/1 -> Add1/1
  Add1/1 -> Gain1/1
  Gain/1 -> Min/1
  Gain1/1 -> Min/2
  Min/1 -> lmd/1

== system AFCToolbox2023a/SimuMoudle/Position-Control/Leader/Subsystem/Follower3/Subsystem/get lmd ==
  Add : Sum  Inputs=+-
  Add1 : Sum  Inputs=+-
  Gain : Gain  Gain=0.707
  Gain1 : Gain  Gain=0.707
  Min : MinMax  Inputs=2
  lmd high : Constant  Value=6.45
  lmd low : Constant  Value=0.45
  v0_max : Constant  Value=3.5
  v0_min : Constant  Value=3
  lmd : Outport
  wires:
  Min/1 -> lmd/1
  Gain1/1 -> Min/2
  Gain/1 -> Min/1
  Add1/1 -> Gain1/1
  lmd high/1 -> Add1/1
  v0_max/1 -> Add1/2
  Add/1 -> Gain/1
  lmd low/1 -> Add/2
  v0_min/1 -> Add/1

== system AFCToolbox2023a/SimuMoudle/UAV/Forces & Moments/Parameters/Air Parameter1/Air Model/H ==
  h : Inport
  1 : Constant
  Add1 : Sum  Inputs=2
  Product4 : Product  Inputs=*/  RndMeth=Zero
  Product5 : Product  Inputs=*/  RndMeth=Zero
  R0 : Constant  Value=6356.766
  H : Outport
  wires:
  Product5/1 -> H/1
  Add1/1 -> Product5/2
  1/1 -> Add1/2
  Product4/1 -> Add1/1
  R0/1 -> Product4/2
  h/1 -> Product5/1, Product4/1

== system AFCToolbox2023a/SimuMoudle/UAV/Forces & Moments/Parameters/Air Parameter1/Air Model/Pressure xishu ==
  note: 9
  note: 1
  note: 2
  note: 3
  note: 4
  note: 5
  note: 6
  note: 7
  note: 8
  Z : Inport
  H : Inport  Port=2
  1 : Switch  Threshold=11.0191  SaturateOnIntegerOverflow=off  InputSameDT=off
  2 : Switch  Threshold=20.0631  SaturateOnIntegerOverflow=off  InputSameDT=off
  3 : Switch  Threshold=32.1619  SaturateOnIntegerOverflow=off  InputSameDT=off
  4 : Switch  Threshold=47.3501  SaturateOnIntegerOverflow=off  InputSameDT=off
  5 : Switch  Threshold=51.4125  SaturateOnIntegerOverflow=off  InputSameDT=off
  6 : Switch  Threshold=71.8020  SaturateOnIntegerOverflow=off  InputSameDT=off
  7 : Switch  Threshold=86  SaturateOnIntegerOverflow=off  InputSameDT=off
  8 : Switch  Threshold=91  SaturateOnIntegerOverflow=off  InputSameDT=off
  Gain : Gain  Gain=1.042e-3
  Gain1 : Gain  Gain=1e-6
  Sum : Sum  Inputs=|++
  constant1 : Constant  Value=2.1671e-4
  constant10 : Constant  Value=8.9155e-4
  constant11 : Constant  Value=2.8338e-3
  constant2 : Constant  Value=0
  constant4 : Constant  Value=1.2274e-5
  constant6 : Constant  Value=2.2730
  constant7 : Constant
  constant8 : Constant  Value=1.1953e-1
  constant9 : Constant  Value=2.5158e-2
  xishu : Outport
  wires:
  Gain1/1 -> 7/1
  Gain/1 -> Sum/2
  H/1 -> Gain/1
  Sum/1 -> Gain1/1
  constant6/1 -> Sum/1
  8/1 -> xishu/1
  7/1 -> 8/3
  constant2/1 -> 8/1
  constant7/1 -> 1/3
  constant8/1 -> 1/1
  constant9/1 -> 2/1
  1/1 -> 2/3
  constant11/1 -> 3/1
  2/1 -> 3/3
  constant10/1 -> 4/1
  3/1 -> 4/3
  constant1/1 -> 5/1
  4/1 -> 5/3
  constant4/1 -> 6/1
  5/1 -> 6/3
  6/1 -> 7/3
  Z/1 -> 2/2, 8/2, 7/2, 6/2, 5/2, 1/2, 3/2, 4/2

== system AFCToolbox2023a/SimuMoudle/UAV/Forces & Moments/Parameters/Air Parameter1/Air Model/T ==
  note: 1
  note: 2
  note: 3
  note: 4
  note: 5
  note: 6
  note: 7
  note: 8
  Z : Inport
  T xishu : Inport  Port=2
  W : Inport  Port=3
  1 : Switch  Threshold=11.0191  SaturateOnIntegerOverflow=off  InputSameDT=off
  2 : Switch  Threshold=20.0631  SaturateOnIntegerOverflow=off  InputSameDT=off
  3 : Switch  Threshold=32.1619  SaturateOnIntegerOverflow=off  InputSameDT=off
  4 : Switch  Threshold=47.3501  SaturateOnIntegerOverflow=off  InputSameDT=off
  5 : Switch  Threshold=51.4125  SaturateOnIntegerOverflow=off  InputSameDT=off
  6 : Switch  Threshold=71.8020  SaturateOnIntegerOverflow=off  InputSameDT=off
  7 : Switch  Threshold=86  SaturateOnIntegerOverflow=off  InputSameDT=off
  Product : Product  RndMeth=Zero
  constant10 : Constant
  constant6 : Constant
  constant8 : Constant
  T : Outport
  wires:
  Product/1 -> T/1
  T xishu/1 -> Product/2
  7/1 -> Product/1
  W/1 -> 3/1, 2/1, 5/1, 6/1, 1/3
  constant8/1 -> 1/1
  1/1 -> 2/3
  2/1 -> 3/3
  constant10/1 -> 4/1
  3/1 -> 4/3
  4/1 -> 5/3
  5/1 -> 6/3
  constant6/1 -> 7/1
  6/1 -> 7/3
  Z/1 -> 2/2, 6/2, 7/2, 5/2, 1/2, 3/2, 4/2

== system AFCToolbox2023a/SimuMoudle/UAV/Forces & Moments/Parameters/Air Parameter1/Air Model/T xishu ==
  note: 8
  note: 7
  note: 6
  note: 5
  note: 4
  note: 3
  note: 2
  note: 1
  Z : Inport
  1 : Switch  Threshold=11.0191  SaturateOnIntegerOverflow=off  InputSameDT=off
  2 : Switch  Threshold=20.0631  SaturateOnIntegerOverflow=off  InputSameDT=off
  3 : Switch  Threshold=32.1619  SaturateOnIntegerOverflow=off  InputSameDT=off
  4 : Switch  Threshold=47.3501  SaturateOnIntegerOverflow=off  InputSameDT=off
  5 : Switch  Threshold=51.4125  SaturateOnIntegerOverflow=off  InputSameDT=off
  6 : Switch  Threshold=71.8020  SaturateOnIntegerOverflow=off  InputSameDT=off
  7 : Switch  Threshold=86  SaturateOnIntegerOverflow=off  InputSameDT=off
  constant1 : Constant  Value=247.021
  constant10 : Constant  Value=270.650
  constant11 : Constant  Value=250.350
  constant4 : Constant  Value=200.590
  constant6 : Constant  Value=186.870
  constant7 : Constant  Value=288.15
  constant8 : Constant  Value=216.650
  constant9 : Constant  Value=221.552
  T xishu : Outport
  wires:
  7/1 -> T xishu/1
  Z/1 -> 4/2, 3/2, 1/2, 5/2, 7/2, 6/2, 2/2
  6/1 -> 7/3
  constant6/1 -> 7/1
  5/1 -> 6/3
  constant4/1 -> 6/1
  4/1 -> 5/3
  constant1/1 -> 5/1
  3/1 -> 4/3
  constant10/1 -> 4/1
  2/1 -> 3/3
  constant11/1 -> 3/1
  1/1 -> 2/3
  constant9/1 -> 2/1
  constant8/1 -> 1/1
  constant7/1 -> 1/3

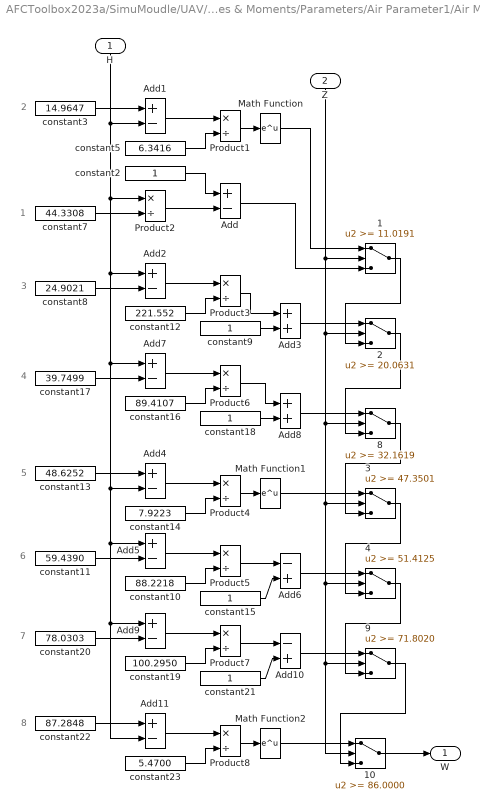
== system AFCToolbox2023a/SimuMoudle/UAV/Forces & Moments/Parameters/Air Parameter1/Air Model/W ==
  note: 8
  note: 7
  note: 4
  note: 6
  note: 5
  note: 3
  note: 2
  note: 1
  H : Inport
  Z : Inport  Port=2
  1 : Switch  Threshold=11.0191  SaturateOnIntegerOverflow=off  InputSameDT=off
  10 : Switch  Threshold=86.0000  SaturateOnIntegerOverflow=off  InputSameDT=off
  2 : Switch  Threshold=20.0631  SaturateOnIntegerOverflow=off  InputSameDT=off
  3 : Switch  Threshold=47.3501  SaturateOnIntegerOverflow=off  InputSameDT=off
  4 : Switch  Threshold=51.4125  SaturateOnIntegerOverflow=off  InputSameDT=off
  8 : Switch  Threshold=32.1619  SaturateOnIntegerOverflow=off  InputSameDT=off
  9 : Switch  Threshold=71.8020  SaturateOnIntegerOverflow=off  InputSameDT=off
  Add{,1..2,4..5,7,9,11} (8 alike) : Sum  Inputs=+-
  Add10 : Sum  Inputs=-+
  Add3 : Sum  Inputs=2
  Add6 : Sum  Inputs=-+
  Add8 : Sum  Inputs=2
  Math Function : Math  SignedPower=on
  Math Function1 : Math  SignedPower=on
  Math Function2 : Math  SignedPower=on
  Product{1..8} (8 alike) : Product  Inputs=*/  RndMeth=Zero
  constant10 : Constant  Value=88.2218
  constant11 : Constant  Value=59.4390
  constant12 : Constant  Value=221.552
  constant13 : Constant  Value=48.6252
  constant14 : Constant  Value=7.9223
  constant{2,9,15,18,21} (5 alike) : Constant
  constant16 : Constant  Value=89.4107
  constant17 : Constant  Value=39.7499
  constant19 : Constant  Value=100.2950
  constant20 : Constant  Value=78.0303
  constant22 : Constant  Value=87.2848
  constant23 : Constant  Value=5.4700
  constant3 : Constant  Value=14.9647
  constant5 : Constant  Value=6.3416
  constant7 : Constant  Value=44.3308
  constant8 : Constant  Value=24.9021
  W : Outport
  wires:
  Z/1 -> 1/2, 2/2, 8/2, 3/2, 4/2, 9/2, 10/2
  10/1 -> W/1
  9/1 -> 10/3
  constant22/1 -> Add11/1
  Math Function2/1 -> 10/1
  Product8/1 -> Math Function2/1
  constant23/1 -> Product8/2
  Add11/1 -> Product8/1
  Add10/1 -> 9/1
  constant21/1 -> Add10/2
  Product7/1 -> Add10/1
  constant20/1 -> Add9/2
  constant19/1 -> Product7/2
  Add9/1 -> Product7/1
  4/1 -> 9/3
  Add7/1 -> Product6/1
  8/1 -> 3/3
  Add8/1 -> 8/1
  constant18/1 -> Add8/2
  Product6/1 -> Add8/1
  constant17/1 -> Add7/2
  constant16/1 -> Product6/2
  2/1 -> 8/3
  Add6/1 -> 4/1
  constant15/1 -> Add6/2
  Product5/1 -> Add6/1
  constant11/1 -> Add5/2
  constant10/1 -> Product5/2
  Add5/1 -> Product5/1
  Math Function1/1 -> 3/1
  Product4/1 -> Math Function1/1
  constant14/1 -> Product4/2
  Add4/1 -> Product4/1
  constant13/1 -> Add4/1
  Add3/1 -> 2/1
  constant9/1 -> Add3/2
  Product3/1 -> Add3/1
  constant8/1 -> Add2/2
  constant12/1 -> Product3/2
  Add2/1 -> Product3/1
  Math Function/1 -> 1/1
  Product1/1 -> Math Function/1
  constant5/1 -> Product1/2
  Add1/1 -> Product1/1
  constant3/1 -> Add1/1
  Product2/1 -> Add/2
  constant2/1 -> Add/1
  constant7/1 -> Product2/2
  Add/1 -> 1/3
  1/1 -> 2/3
  3/1 -> 4/3
  H/1 -> Add7/1, Add11/2, Add9/1, Add5/1, Add4/2, Add2/1, Product2/1, Add1/2

== system AFCToolbox2023a/SimuMoudle/UAV/Forces & Moments/Parameters/Air Parameter1/Air Model/W zhishu ==
  note: 1
  note: 2
  note: 3
  note: 4
  note: 5
  note: 6
  note: 7
  note: 8
  Z : Inport
  1 : Switch  Threshold=11.0191  SaturateOnIntegerOverflow=off  InputSameDT=off
  2 : Switch  Threshold=20.0631  SaturateOnIntegerOverflow=off  InputSameDT=off
  3 : Switch  Threshold=32.1619  SaturateOnIntegerOverflow=off  InputSameDT=off
  4 : Switch  Threshold=47.3501  SaturateOnIntegerOverflow=off  InputSameDT=off
  5 : Switch  Threshold=51.4125  SaturateOnIntegerOverflow=off  InputSameDT=off
  6 : Switch  Threshold=71.8020  SaturateOnIntegerOverflow=off  InputSameDT=off
  7 : Switch  Threshold=86  SaturateOnIntegerOverflow=off  InputSameDT=off
  constant1 : Constant  Value=11.2011
  constant10 : Constant
  constant11 : Constant  Value=-13.2011
  constant4 : Constant  Value=16.0816
  constant6 : Constant
  constant7 : Constant  Value=4.2559
  constant8 : Constant
  constant9 : Constant  Value=-35.1629
  zhishu : Outport
  wires:
  constant7/1 -> 1/3
  constant8/1 -> 1/1
  constant9/1 -> 2/1
  1/1 -> 2/3
  constant11/1 -> 3/1
  2/1 -> 3/3
  constant10/1 -> 4/1
  3/1 -> 4/3
  constant1/1 -> 5/1
  4/1 -> 5/3
  constant4/1 -> 6/1
  5/1 -> 6/3
  constant6/1 -> 7/1
  6/1 -> 7/3
  Z/1 -> 2/2, 6/2, 7/2, 5/2, 1/2, 3/2, 4/2
  7/1 -> zhishu/1

== system AFCToolbox2023a/SimuMoudle/UAV/Forces & Moments/Parameters/Air Parameter1/Air Model/W zhishu1 ==
  note: 8
  note: 7
  note: 6
  note: 5
  note: 4
  note: 3
  note: 2
  note: 1
  Z : Inport
  1 : Switch  Threshold=11.0191  SaturateOnIntegerOverflow=off  InputSameDT=off
  2 : Switch  Threshold=20.0631  SaturateOnIntegerOverflow=off  InputSameDT=off
  3 : Switch  Threshold=32.1619  SaturateOnIntegerOverflow=off  InputSameDT=off
  4 : Switch  Threshold=47.3501  SaturateOnIntegerOverflow=off  InputSameDT=off
  5 : Switch  Threshold=51.4125  SaturateOnIntegerOverflow=off  InputSameDT=off
  6 : Switch  Threshold=71.8020  SaturateOnIntegerOverflow=off  InputSameDT=off
  7 : Switch  Threshold=86  SaturateOnIntegerOverflow=off  InputSameDT=off
  constant1 : Constant  Value=12.2011
  constant10 : Constant
  constant11 : Constant  Value=-12.2011
  constant4 : Constant  Value=17.0816
  constant6 : Constant
  constant7 : Constant  Value=5.2559
  constant8 : Constant
  constant9 : Constant  Value=-34.1629
  zhishu : Outport
  wires:
  7/1 -> zhishu/1
  Z/1 -> 4/2, 3/2, 1/2, 5/2, 7/2, 6/2, 2/2
  6/1 -> 7/3
  constant6/1 -> 7/1
  5/1 -> 6/3
  constant4/1 -> 6/1
  4/1 -> 5/3
  constant1/1 -> 5/1
  3/1 -> 4/3
  constant10/1 -> 4/1
  2/1 -> 3/3
  constant11/1 -> 3/1
  1/1 -> 2/3
  constant9/1 -> 2/1
  constant8/1 -> 1/1
  constant7/1 -> 1/3

== system AFCToolbox2023a/SimuMoudle/UAV/Forces & Moments/Parameters/Air Parameter1/Air Model/rho xishu ==
  note: 8
  note: 7
  note: 6
  note: 5
  note: 4
  note: 3
  note: 2
  note: 1
  note: 9
  Z : Inport
  1 : Switch  Threshold=11.0191  SaturateOnIntegerOverflow=off  InputSameDT=off
  2 : Switch  Threshold=20.0631  SaturateOnIntegerOverflow=off  InputSameDT=off
  3 : Switch  Threshold=32.1619  SaturateOnIntegerOverflow=off  InputSameDT=off
  4 : Switch  Threshold=47.3501  SaturateOnIntegerOverflow=off  InputSameDT=off
  5 : Switch  Threshold=51.4125  SaturateOnIntegerOverflow=off  InputSameDT=off
  6 : Switch  Threshold=71.8020  SaturateOnIntegerOverflow=off  InputSameDT=off
  7 : Switch  Threshold=86  SaturateOnIntegerOverflow=off  InputSameDT=off
  8 : Switch  Threshold=91  SaturateOnIntegerOverflow=off  InputSameDT=off
  constant1 : Constant  Value=2.5280e-4
  constant10 : Constant  Value=9.4920e-4
  constant11 : Constant  Value=3.2618e-3
  constant2 : Constant  Value=0
  constant4 : Constant  Value=1.7632e-5
  constant6 : Constant  Value=3.6411e-6
  constant7 : Constant
  constant8 : Constant  Value=1.5898e-1
  constant9 : Constant  Value=3.2722e-2
  xishu : Outport
  wires:
  Z/1 -> 4/2, 3/2, 1/2, 5/2, 6/2, 7/2, 8/2, 2/2
  6/1 -> 7/3
  constant6/1 -> 7/1
  5/1 -> 6/3
  constant4/1 -> 6/1
  4/1 -> 5/3
  constant1/1 -> 5/1
  3/1 -> 4/3
  constant10/1 -> 4/1
  2/1 -> 3/3
  constant11/1 -> 3/1
  1/1 -> 2/3
  constant9/1 -> 2/1
  constant8/1 -> 1/1
  constant7/1 -> 1/3
  constant2/1 -> 8/1
  7/1 -> 8/3
  8/1 -> xishu/1

== system AFCToolbox2023a/基础导航算法模型库/ECL EKF/init_state/State_mag1/Subsystem1/Subsystem/round down1 ==
  lat : Inport
  Data Type Conversion2 : DataTypeConversion  OutDataTypeStr=single  SaturateOnIntegerOverflow=off  RndMeth=Floor
  Floor2 : Rounding
  rad_to_index2 : Gain  Gain=0.1  OutDataTypeStr=int32
  rad_to_index3 : Gain  Gain=10  OutDataTypeStr=int32
  min_lat : Outport
  wires:
  Floor2/1 -> rad_to_index3/1
  lat/1 -> rad_to_index2/1
  rad_to_index3/1 -> min_lat/1
  rad_to_index2/1 -> Data Type Conversion2/1
  Data Type Conversion2/1 -> Floor2/1

== system AFCToolbox2023a/基础导航算法模型库/ECL EKF/init_state/State_mag1/Subsystem1/Subsystem/round down3 ==
  lon : Inport
  Data Type Conversion2 : DataTypeConversion  OutDataTypeStr=single  SaturateOnIntegerOverflow=off  RndMeth=Floor
  Floor2 : Rounding
  rad_to_index2 : Gain  Gain=0.1  OutDataTypeStr=int32
  rad_to_index3 : Gain  Gain=10  OutDataTypeStr=int32
  min_lon : Outport
  wires:
  Floor2/1 -> rad_to_index3/1
  rad_to_index3/1 -> min_lon/1
  rad_to_index2/1 -> Data Type Conversion2/1
  lon/1 -> rad_to_index2/1
  Data Type Conversion2/1 -> Floor2/1

== system AFCToolbox2023a/基础导航算法模型库/ECL EKF/init_state/State_mag1/Subsystem1/Subsystem2/round down1 ==
  lat : Inport
  Data Type Conversion2 : DataTypeConversion  OutDataTypeStr=single  SaturateOnIntegerOverflow=off  RndMeth=Floor
  Floor2 : Rounding
  rad_to_index2 : Gain  Gain=0.1  OutDataTypeStr=int32
  rad_to_index3 : Gain  Gain=10  OutDataTypeStr=int32
  min_lat : Outport
  wires:
  Data Type Conversion2/1 -> Floor2/1
  rad_to_index2/1 -> Data Type Conversion2/1
  rad_to_index3/1 -> min_lat/1
  lat/1 -> rad_to_index2/1
  Floor2/1 -> rad_to_index3/1

== system AFCToolbox2023a/基础导航算法模型库/ECL EKF/init_state/State_mag1/Subsystem1/Subsystem2/round down3 ==
  lon : Inport
  Data Type Conversion2 : DataTypeConversion  OutDataTypeStr=single  SaturateOnIntegerOverflow=off  RndMeth=Floor
  Floor2 : Rounding
  rad_to_index2 : Gain  Gain=0.1  OutDataTypeStr=int32
  rad_to_index3 : Gain  Gain=10  OutDataTypeStr=int32
  min_lon : Outport
  wires:
  Data Type Conversion2/1 -> Floor2/1
  lon/1 -> rad_to_index2/1
  rad_to_index2/1 -> Data Type Conversion2/1
  rad_to_index3/1 -> min_lon/1
  Floor2/1 -> rad_to_index3/1

== system AFCToolbox2023a/基础导航算法模型库/ECL EKF/init_state/State_mag1/Subsystem1/Subsystem3/round down1 ==
  lat : Inport
  Data Type Conversion2 : DataTypeConversion  OutDataTypeStr=single  SaturateOnIntegerOverflow=off  RndMeth=Floor
  Floor2 : Rounding
  rad_to_index2 : Gain  Gain=0.1  OutDataTypeStr=int32
  rad_to_index3 : Gain  Gain=10  OutDataTypeStr=int32
  min_lat : Outport
  wires:
  Data Type Conversion2/1 -> Floor2/1
  rad_to_index2/1 -> Data Type Conversion2/1
  rad_to_index3/1 -> min_lat/1
  lat/1 -> rad_to_index2/1
  Floor2/1 -> rad_to_index3/1

== system AFCToolbox2023a/基础导航算法模型库/ECL EKF/init_state/State_mag1/Subsystem1/Subsystem3/round down3 ==
  lon : Inport
  Data Type Conversion2 : DataTypeConversion  OutDataTypeStr=single  SaturateOnIntegerOverflow=off  RndMeth=Floor
  Floor2 : Rounding
  rad_to_index2 : Gain  Gain=0.1  OutDataTypeStr=int32
  rad_to_index3 : Gain  Gain=10  OutDataTypeStr=int32
  min_lon : Outport
  wires:
  Data Type Conversion2/1 -> Floor2/1
  lon/1 -> rad_to_index2/1
  rad_to_index2/1 -> Data Type Conversion2/1
  rad_to_index3/1 -> min_lon/1
  Floor2/1 -> rad_to_index3/1
